simulink model "DualBuckPPS22016"  (R2024b)
settings: Solver=ode45  StartTime=0.0  StopTime=0.5  RelTol=1e-3
model workspace (MAT data in the model file):
  D = 50
  T = 0.0333333333333
undefined symbols (not defined in the file): D_T_DOWN_Given, D_T_UP_Given, DiscIntNeverNeededParam, P, T_pulse, TP
libraries: spsOnDelayLib x30, dspsnks4 x12, dspfdesign x11, spsCurrentMeasurementLib x11, spsSeriesRLCBranchLib x6, spsMosfetLib x4, slpidlib x4, spsVoltageMeasurementLib x4, simulink x3, spsControlledCurrentSourceLib x1, spsDCVoltageSourceLib x1, spspowerguiLib x1
(part 1 of 2)
settings Model: SimulationMode=accelerator  Creator=10474  LastModifiedBy=admin
settings SolverCC: AlgebraicLoopSolver=TrustRegion
settings OptimizationCC: ReuseModelBlockBuffer=off
settings DebuggingCC: UnconnectedInputMsg=warning  UnconnectedOutputMsg=warning  UnconnectedLineMsg=warning  ArithmeticOperatorsInVariantConditions=warning
settings ModelReferenceCC: EnableRefExpFcnMdlSchedulingChecks=on
settings SFSimCC: CustomCodeUndefinedFunction=UseInterfaceOnly
settings RTWCC: GPUComputeCapability=3.5
settings CodeAppCC: StateflowObjectComments=on

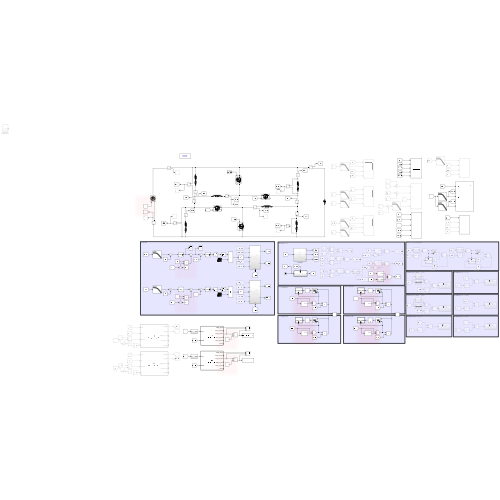
[thumbnail: Simulink's stored preview of the top-level diagram]
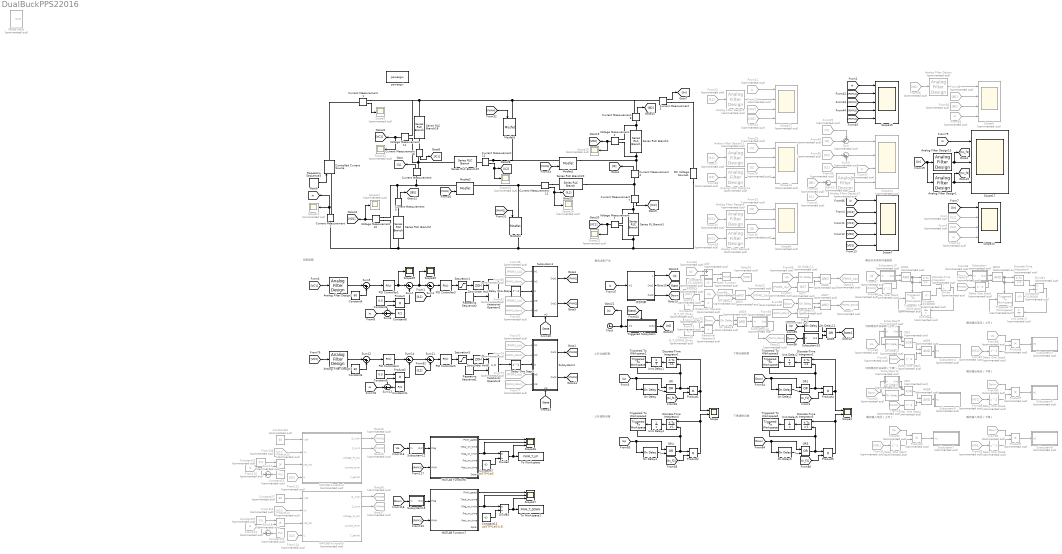
== system DualBuckPPS22016 ==
  note: 控制回路
  note: 上升尖峰获取
  note: 上升滤除尖峰
  note: 下降尖峰获取
  note: 下降滤除尖峰
  note: 瞬态输出电压（上升）
  note: 切回稳态开关采样（上升）
  note: 瞬态输入电压（上升）
  note: 瞬态输入电压（下降）
  note: 瞬态开关序列均值获取
  note: 瞬态输出电压（下降）
  note: 切回稳态开关采样（下降）
  note: 瞬态波形产生
  AND{1..8} (8 alike) : Logic  Commented=on  IconShape=distinctive  AllPortsSameDT=off  OutDataTypeStr=boolean
  AND9 : Logic  Operator=OR  IconShape=distinctive  AllPortsSameDT=off  OutDataTypeStr=boolean
  Add : Sum  Commented=on  Inputs=+-
  Analog Filter Design{,5..6,9..12} (7 alike) : dspfdesign/Analog Filter Design  Commented=on  method=Butterworth  filttype=Lowpass  N=8  Wlo=2*pi*5000  Whi=80  Rp=2  Rs=40
  Analog Filter Design1 : dspfdesign/Analog Filter Design  method=Butterworth  filttype=Lowpass  N=2  Wlo=2*pi*2500  Whi=80  Rp=2  Rs=40
  Analog Filter Design13 : dspfdesign/Analog Filter Design  method=Butterworth  filttype=Lowpass  N=2  Wlo=2*pi*10000  Whi=80  Rp=2  Rs=40
  Analog Filter Design2 : dspfdesign/Analog Filter Design  method=Butterworth  filttype=Lowpass  N=1  Wlo=10  Whi=80  Rp=2  Rs=40
  Analog Filter Design3 : dspfdesign/Analog Filter Design  method=Butterworth  filttype=Lowpass  N=1  Wlo=10  Whi=80  Rp=2  Rs=40
  Clock : Clock
  Constant : Constant  Commented=on  Value=1/100000
  Constant1 : Constant  Commented=on  Value=1/100000
  Constant10 : Constant  Commented=on  Value=D_T_DOWN_Given
  Constant11 : Constant  Value=P/2
  Constant12 : Constant  Value=ceil(TP*1e5-0.5)
  Constant2 : Constant  Commented=on  Value=D_T_UP_Given
  Constant22 : Constant  Commented=on  Value=0.5
  Constant23 : Constant  Commented=on  Value=P/2
  Constant24 : Constant  Commented=on  Value=60
  Constant25 : Constant  Commented=on  Value=0.5
  Constant26 : Constant  Commented=on  Value=P/2
  Constant27 : Constant  Commented=on  Value=60
  Constant3 : Constant  Value=60
  Constant4 : Constant  Value=60
  Constant5 : Constant  Commented=on  Value=1/100000
  Constant6 : Constant  Value=0.5
  Constant7 : Constant  Value=ceil(TP*1e5)
  Constant8 : Constant  Value=P/2
  Constant9 : Constant  Value=0.5
  Controlled Current Source : spsControlledCurrentSourceLib/Controlled Current Source  Initialize=on  Source_Type=DC  Amplitude=0  Phase=0  Frequency=0  Measurements=None
  Current Measurement{,1..8,11..12} (11 alike) : spsCurrentMeasurementLib/Current Measurement  PhasorSimulation=off  OutputType=Complex  PSBequivalent=0
  DC Voltage Source1 : spsDCVoltageSourceLib/DC Voltage Source  Amplitude=270  Measurements=None
  Delay One Step : Delay  DelayLength=1
  Delay One Step1 : Delay  Commented=on
  Delay One Step{2..3,5..8} (6 alike) : Delay  Commented=on  DelayLength=1
  Delay One Step4 : Delay  Commented=on
  Delay One Step9 : Delay  DelayLength=1
  Discrete-Time Integrator : DiscreteIntegrator  Commented=on  ExternalReset=falling  SampleTime=-1  ICPrevOutput=DiscIntNeverNeededParam  ICPrevScaledInput=DiscIntNeverNeededParam
  Discrete-Time Integrator{1..2,4..5} (4 alike) : DiscreteIntegrator  ExternalReset=falling  SampleTime=-1  ICPrevOutput=DiscIntNeverNeededParam  ICPrevScaledInput=DiscIntNeverNeededParam
  Discrete-Time Integrator3 : DiscreteIntegrator  Commented=on  ExternalReset=falling  SampleTime=-1  ICPrevOutput=DiscIntNeverNeededParam  ICPrevScaledInput=DiscIntNeverNeededParam
  Divide : Product  Commented=on  Inputs=*/
  Divide1 : Product  Commented=on  Inputs=*/
  Divide2 : Product  Inputs=*/
  Divide3 : Product  Inputs=*/
  From{,22,27,36,111} (5 alike) : From  Commented=on  GotoTag=IL1
  From{10,55,61,66} (4 alike) : From  Commented=on  GotoTag=PWM1
  From109 : From  Commented=on  GotoTag=VC1
  From{14,21,37,39,110,113} (6 alike) : From  Commented=on  GotoTag=io  TagVisibility=global
  From112 : From  Commented=on  GotoTag=VC2
  From{9,28,35,114} (4 alike) : From  Commented=on  GotoTag=IL2
  From{15,25,29,41} (4 alike) : From  Commented=on  GotoTag=I1
  From16 : From  Commented=on  GotoTag=I2
  From17 : From  Commented=on  GotoTag=IC1
  From18 : From  Commented=on  GotoTag=IC2
  From23 : From  Commented=on  GotoTag=VC2
  From24 : From  Commented=on  GotoTag=VG2
  From26 : From  Commented=on  GotoTag=I2
  From34 : From  Commented=on  GotoTag=I2
  From38 : From  Commented=on  GotoTag=IB2
  From40 : From  Commented=on  GotoTag=IB1
  From46 : From  Commented=on  GotoTag=IB1
  From48 : From  Commented=on  GotoTag=IB1
  From49 : From  Commented=on  GotoTag=PWM1_Up
  From50 : From  Commented=on  GotoTag=PWM1_Down
  From51 : From  Commented=on  GotoTag=PWM2_Up
  From{56,67..69,89,92} (6 alike) : From  Commented=on  GotoTag=Up  TagVisibility=global
  From57 : From  Commented=on  GotoTag=PWM1_Up
  From{58,60,72,82,90,94} (6 alike) : From  Commented=on  GotoTag=Down  TagVisibility=global
  From59 : From  Commented=on  GotoTag=PWM1_Down
  From62 : From  Commented=on  GotoTag=PWM2_Down
  From63 : From  Commented=on  GotoTag=t0
  From65 : From  Commented=on  GotoTag=t
  From70 : From  Commented=on  GotoTag=PWM1_Up
  From71 : From  Commented=on  GotoTag=MW
  From73 : From  Commented=on  GotoTag=MW
  From74 : From  Commented=on  GotoTag=PWM1_Down
  From75 : From  Commented=on  GotoTag=PWM2_Up
  From77 : From  Commented=on  GotoTag=PWM2_Down
  From87 : From  Commented=on  GotoTag=VC1
  From88 : From  Commented=on  GotoTag=VC1
  From91 : From  Commented=on  GotoTag=VG1
  From93 : From  Commented=on  GotoTag=VG1
  Goto16 : Goto  Commented=on  GotoTag=PWM2_Up
  Goto17 : Goto  Commented=on  GotoTag=PWM2_Down
  Goto22 : Goto  Commented=on  GotoTag=PWM1_Down
  Goto23 : Goto  Commented=on  GotoTag=PWM1_Up
  Goto24 : Goto  Commented=on  GotoTag=MW
  Goto25 : Goto  Commented=on  GotoTag=PWM1
  Goto26 : Goto  Commented=on  GotoTag=PWM2
  Goto36 : Goto  Commented=on  GotoTag=PWM3
  Goto37 : Goto  Commented=on  GotoTag=PWM4
  MATLAB Function4 : MATLAB Function  Commented=on  TreatAsAtomicUnit=on
  MATLAB Function5 : MATLAB Function  Commented=on  TreatAsAtomicUnit=on
  MATLAB Function6 : MATLAB Function  TreatAsAtomicUnit=on
  MATLAB Function7 : MATLAB Function  TreatAsAtomicUnit=on
  Math Function : Math  Commented=on  Operator=mod
  Mosfet{1..4} (4 alike) : spsMosfetLib/Mosfet  Ron=53e-3  Lon=0  Rd=0.001  Vfd=2  IC=0  Rs=1e5  Cs=inf  Measurements=on
  NOT7 : Logic  Commented=on  Operator=NOT  IconShape=distinctive  AllPortsSameDT=off  OutDataTypeStr=boolean
  NOT8 : Logic  Commented=on  Operator=NOT  IconShape=distinctive  AllPortsSameDT=off  OutDataTypeStr=boolean
  OR{,1,4..5} (4 alike) : Logic  Operator=OR  IconShape=distinctive  AllPortsSameDT=off  OutDataTypeStr=boolean
  OR2 : Logic  Commented=on  Operator=XOR  IconShape=distinctive  AllPortsSameDT=off  OutDataTypeStr=boolean
  OR3 : Logic  Commented=on  Operator=XOR  IconShape=distinctive  AllPortsSameDT=off  OutDataTypeStr=boolean
  On Delay{,1,4..5} (4 alike) : spsOnDelayLib/On Delay  DelayType=Off delay  delay=TP  ic=0  Ts=0
  On Delay10 : spsOnDelayLib/On Delay  Commented=on  DelayType=Off delay  delay=ceil((TP-(ceil(TP*1e5)*1e-5-TP))*1e5)*1e-5-(TP-(ceil(TP*1e5)*1e-5-TP))  ic=0  Ts=0
  On Delay11 : spsOnDelayLib/On Delay  DelayType=Off delay  delay=ceil(TP*1e5)*1e-5-TP  ic=0  Ts=0
  On Delay12 : spsOnDelayLib/On Delay  Commented=on  DelayType=Off delay  delay=ceil(TP*1e5)*1e-5-TP  ic=0  Ts=0
  On Delay2 : spsOnDelayLib/On Delay  Commented=on  DelayType=Off delay  delay=ceil(TP*1e5)*1e-5-TP  ic=0  Ts=0
  On Delay3 : spsOnDelayLib/On Delay  Commented=on  DelayType=Off delay  delay=30e-6  ic=0  Ts=0
  On Delay8 : spsOnDelayLib/On Delay  Commented=on  DelayType=Off delay  delay=ceil((TP-(ceil(TP*1e5)*1e-5-TP))*1e5)*1e-5-(TP-(ceil(TP*1e5)*1e-5-TP))  ic=0  Ts=0
  On Delay9 : spsOnDelayLib/On Delay  Commented=on  DelayType=Off delay  delay=30e-6  ic=0  Ts=0
  PID Controller1 : slpidlib/PID Controller  Controller=PI  Form=Parallel  TimeDomain=Discrete-time  UseExternalTs=off  SampleTime=-1  IntegratorMethod=Forward Euler  FilterMethod=Forward Euler  ControllerParametersSource=internal  P=0.15  I=0.5  UseKiTs=off  D=0  UseExternalDerivativeSource=off  N=100  UseFilter=on  TunerSelectOption=Transfer Function Based (PID Tuner App)  InitialConditionSource=internal  InitialConditionForIntegrator=0  InitialConditionForFilter=0  DifferentiatorICPrevScaledInput=0  ExternalReset=none  TrackingMode=off  Kt=1  LimitOutput=on  SatLimitsSource=internal  UpperSaturationLimit=10  LowerSaturationLimit=-10  LinearizeAsGain=on  AntiWindupMode=none  Kb=1  LimitIntegrator=off  UpperIntegratorSaturationLimit=inf  LowerIntegratorSaturationLimit=-inf  POutMin=[]  POutMax=[]  IOutMin=[]  IOutMax=[]  DOutMin=[]  DOutMax=[]  NOutMin=[]  NOutMax=[]  SumOutMin=[]  SumOutMax=[]  SaturationOutMin=[]  SaturationOutMax=[]  PParamMin=[]  PParamMax=[]  IParamMin=[]  IParamMax=[]  DParamMin=[]  DParamMax=[]  NParamMin=[]  NParamMax=[]  KbParamMin=[]  KbParamMax=[]  KtParamMin=[]  KtParamMax=[]  KbOutMin=[]  KbOutMax=[]  KtOutMin=[]  KtOutMax=[]  IntegratorOutMin=[]  IntegratorOutMax=[]  FilterOutMin=[]  FilterOutMax=[]  SumI1OutMin=[]  SumI1OutMax=[]  SumI2OutMin=[]  SumI2OutMax=[]  SumI3OutMin=[]  SumI3OutMax=[]  SumI4OutMin=[]  SumI4OutMax=[]  SumDOutMin=[]  SumDOutMax=[]  DifferentiatorOutMin=[]  DifferentiatorOutMax=[]  FilterDiffOutCoefMin=[]  FilterDiffOutCoefMax=[]  ReciprocalOutMin=[]  ReciprocalOutMax=[]  SumDenOutMin=[]  SumDenOutMax=[]  SumNumOutMin=[]  SumNumOutMax=[]  DivideOutMin=[]  DivideOutMax=[]  UdiffTsProdOutMin=[]  UdiffTsProdOutMax=[]  NTsProdOutMin=[]  NTsProdOutMax=[]  UintegralTsProdOutMin=[]  UintegralTsProdOutMax=[]  UngainTsProdOutMin=[]  UngainTsProdOutMax=[]  ClampingZeroOutDataTypeStr=Inherit: Inherit via back propagation  ClampingZeroOutMin=[]  ClampingZeroOutMax=[]  FilterDenConstantOutDataTypeStr=Inherit: Inherit via back propagation  FilterDenConstantOutMin=[]  FilterDenConstantOutMax=[]  PCopyOutDataTypeStr=Inherit: Inherit via back propagation  PCopyOutMin=[]  PCopyOutMax=[]  NCopyOutDataTypeStr=Inherit: Inherit via back propagation  NCopyOutMin=[]  NCopyOutMax=[]  IntegratorContinuousStateAttributes=''  IntegratorStateMustResolveToSignalObject=off  IntegratorRTWStateStorageClass=Auto  FilterContinuousStateAttributes=''  FilterStateMustResolveToSignalObject=off  FilterRTWStateStorageClass=Auto  ParallelPVariant=InternalParameters  IdealPVariant=Disabled  IVariant=InternalParameters  DVariant=Disabled  IntegratorVariant=Discrete  SatVariant=Enabled  AWVariant=Passthrough  PCopyVariant=Disabled  TRVariant=Disabled  FdbkBlocksVariant=Forward  IdealPFdbkVariant=Disabled  SatFdbkVariant=Disabled  DerivativeFilterVariant=Disabled  NVariant=Disabled  NCopyVariant=Disabled_SignalSpec  FilterICVariant=Disabled  IntegratorICVariant=InternalICs  ExternalResetVariant=Disabled  TRSumVariant=Passthrough  SumFdbkVariant=Disabled  SumVariant=Sum_PI  TsampFilterVariant=InternalTs  TsampNgainVariant=Passthrough  TsampIntegralVariant=Disabled_SignalSpec  ExternalSaturationOutDataTypeStr=Inherit: Same as second input  DerivativeSourceVariant=Disabled  PreIntVariant=InternalPreInt
  PID Controller3 : slpidlib/PID Controller  Controller=PI  Form=Parallel  TimeDomain=Discrete-time  UseExternalTs=off  SampleTime=-1  IntegratorMethod=Forward Euler  FilterMethod=Forward Euler  ControllerParametersSource=internal  P=0.2  I=2  UseKiTs=off  D=0  UseExternalDerivativeSource=off  N=100  UseFilter=on  TunerSelectOption=Transfer Function Based (PID Tuner App)  InitialConditionSource=internal  InitialConditionForIntegrator=0  InitialConditionForFilter=0  DifferentiatorICPrevScaledInput=0  ExternalReset=none  TrackingMode=off  Kt=1  LimitOutput=on  SatLimitsSource=internal  UpperSaturationLimit=0.98  LowerSaturationLimit=0  LinearizeAsGain=on  AntiWindupMode=none  Kb=1  LimitIntegrator=off  UpperIntegratorSaturationLimit=inf  LowerIntegratorSaturationLimit=-inf  POutMin=[]  POutMax=[]  IOutMin=[]  IOutMax=[]  DOutMin=[]  DOutMax=[]  NOutMin=[]  NOutMax=[]  SumOutMin=[]  SumOutMax=[]  SaturationOutMin=[]  SaturationOutMax=[]  PParamMin=[]  PParamMax=[]  IParamMin=[]  IParamMax=[]  DParamMin=[]  DParamMax=[]  NParamMin=[]  NParamMax=[]  KbParamMin=[]  KbParamMax=[]  KtParamMin=[]  KtParamMax=[]  KbOutMin=[]  KbOutMax=[]  KtOutMin=[]  KtOutMax=[]  IntegratorOutMin=[]  IntegratorOutMax=[]  FilterOutMin=[]  FilterOutMax=[]  SumI1OutMin=[]  SumI1OutMax=[]  SumI2OutMin=[]  SumI2OutMax=[]  SumI3OutMin=[]  SumI3OutMax=[]  SumI4OutMin=[]  SumI4OutMax=[]  SumDOutMin=[]  SumDOutMax=[]  DifferentiatorOutMin=[]  DifferentiatorOutMax=[]  FilterDiffOutCoefMin=[]  FilterDiffOutCoefMax=[]  ReciprocalOutMin=[]  ReciprocalOutMax=[]  SumDenOutMin=[]  SumDenOutMax=[]  SumNumOutMin=[]  SumNumOutMax=[]  DivideOutMin=[]  DivideOutMax=[]  UdiffTsProdOutMin=[]  UdiffTsProdOutMax=[]  NTsProdOutMin=[]  NTsProdOutMax=[]  UintegralTsProdOutMin=[]  UintegralTsProdOutMax=[]  UngainTsProdOutMin=[]  UngainTsProdOutMax=[]  ClampingZeroOutDataTypeStr=Inherit: Inherit via back propagation  ClampingZeroOutMin=[]  ClampingZeroOutMax=[]  FilterDenConstantOutDataTypeStr=Inherit: Inherit via back propagation  FilterDenConstantOutMin=[]  FilterDenConstantOutMax=[]  PCopyOutDataTypeStr=Inherit: Inherit via back propagation  PCopyOutMin=[]  PCopyOutMax=[]  NCopyOutDataTypeStr=Inherit: Inherit via back propagation  NCopyOutMin=[]  NCopyOutMax=[]  IntegratorContinuousStateAttributes=''  IntegratorStateMustResolveToSignalObject=off  IntegratorRTWStateStorageClass=Auto  FilterContinuousStateAttributes=''  FilterStateMustResolveToSignalObject=off  FilterRTWStateStorageClass=Auto  ParallelPVariant=InternalParameters  IdealPVariant=Disabled  IVariant=InternalParameters  DVariant=Disabled  IntegratorVariant=Discrete  SatVariant=Enabled  AWVariant=Passthrough  PCopyVariant=Disabled  TRVariant=Disabled  FdbkBlocksVariant=Forward  IdealPFdbkVariant=Disabled  SatFdbkVariant=Disabled  DerivativeFilterVariant=Disabled  NVariant=Disabled  NCopyVariant=Disabled_SignalSpec  FilterICVariant=Disabled  IntegratorICVariant=InternalICs  ExternalResetVariant=Disabled  TRSumVariant=Passthrough  SumFdbkVariant=Disabled  SumVariant=Sum_PI  TsampFilterVariant=InternalTs  TsampNgainVariant=Passthrough  TsampIntegralVariant=Disabled_SignalSpec  ExternalSaturationOutDataTypeStr=Inherit: Same as second input  DerivativeSourceVariant=Disabled  PreIntVariant=InternalPreInt
  PID Controller4 : slpidlib/PID Controller  Controller=PI  Form=Parallel  TimeDomain=Discrete-time  UseExternalTs=off  SampleTime=-1  IntegratorMethod=Forward Euler  FilterMethod=Forward Euler  ControllerParametersSource=internal  P=0.15  I=0.5  UseKiTs=off  D=0  UseExternalDerivativeSource=off  N=100  UseFilter=on  TunerSelectOption=Transfer Function Based (PID Tuner App)  InitialConditionSource=internal  InitialConditionForIntegrator=0  InitialConditionForFilter=0  DifferentiatorICPrevScaledInput=0  ExternalReset=none  TrackingMode=off  Kt=1  LimitOutput=off  SatLimitsSource=internal  UpperSaturationLimit=1  LowerSaturationLimit=-1  LinearizeAsGain=on  AntiWindupMode=none  Kb=1  LimitIntegrator=off  UpperIntegratorSaturationLimit=inf  LowerIntegratorSaturationLimit=-inf  POutMin=[]  POutMax=[]  IOutMin=[]  IOutMax=[]  DOutMin=[]  DOutMax=[]  NOutMin=[]  NOutMax=[]  SumOutMin=[]  SumOutMax=[]  SaturationOutMin=[]  SaturationOutMax=[]  PParamMin=[]  PParamMax=[]  IParamMin=[]  IParamMax=[]  DParamMin=[]  DParamMax=[]  NParamMin=[]  NParamMax=[]  KbParamMin=[]  KbParamMax=[]  KtParamMin=[]  KtParamMax=[]  KbOutMin=[]  KbOutMax=[]  KtOutMin=[]  KtOutMax=[]  IntegratorOutMin=[]  IntegratorOutMax=[]  FilterOutMin=[]  FilterOutMax=[]  SumI1OutMin=[]  SumI1OutMax=[]  SumI2OutMin=[]  SumI2OutMax=[]  SumI3OutMin=[]  SumI3OutMax=[]  SumI4OutMin=[]  SumI4OutMax=[]  SumDOutMin=[]  SumDOutMax=[]  DifferentiatorOutMin=[]  DifferentiatorOutMax=[]  FilterDiffOutCoefMin=[]  FilterDiffOutCoefMax=[]  ReciprocalOutMin=[]  ReciprocalOutMax=[]  SumDenOutMin=[]  SumDenOutMax=[]  SumNumOutMin=[]  SumNumOutMax=[]  DivideOutMin=[]  DivideOutMax=[]  UdiffTsProdOutMin=[]  UdiffTsProdOutMax=[]  NTsProdOutMin=[]  NTsProdOutMax=[]  UintegralTsProdOutMin=[]  UintegralTsProdOutMax=[]  UngainTsProdOutMin=[]  UngainTsProdOutMax=[]  ClampingZeroOutDataTypeStr=Inherit: Inherit via back propagation  ClampingZeroOutMin=[]  ClampingZeroOutMax=[]  FilterDenConstantOutDataTypeStr=Inherit: Inherit via back propagation  FilterDenConstantOutMin=[]  FilterDenConstantOutMax=[]  PCopyOutDataTypeStr=Inherit: Inherit via back propagation  PCopyOutMin=[]  PCopyOutMax=[]  NCopyOutDataTypeStr=Inherit: Inherit via back propagation  NCopyOutMin=[]  NCopyOutMax=[]  IntegratorContinuousStateAttributes=''  IntegratorStateMustResolveToSignalObject=off  IntegratorRTWStateStorageClass=Auto  FilterContinuousStateAttributes=''  FilterStateMustResolveToSignalObject=off  FilterRTWStateStorageClass=Auto  ParallelPVariant=InternalParameters  IdealPVariant=Disabled  IVariant=InternalParameters  DVariant=Disabled  IntegratorVariant=Discrete  SatVariant=Disabled  AWVariant=Passthrough  PCopyVariant=Disabled  TRVariant=Disabled  FdbkBlocksVariant=Forward  IdealPFdbkVariant=Disabled  SatFdbkVariant=Disabled  DerivativeFilterVariant=Disabled  NVariant=Disabled  NCopyVariant=Disabled_SignalSpec  FilterICVariant=Disabled  IntegratorICVariant=InternalICs  ExternalResetVariant=Disabled  TRSumVariant=Passthrough  SumFdbkVariant=Disabled  SumVariant=Sum_PI  TsampFilterVariant=InternalTs  TsampNgainVariant=Passthrough  TsampIntegralVariant=Disabled_SignalSpec  ExternalSaturationOutDataTypeStr=Inherit: Same as second input  DerivativeSourceVariant=Disabled  PreIntVariant=InternalPreInt
  PID Controller5 : slpidlib/PID Controller  Controller=PI  Form=Parallel  TimeDomain=Discrete-time  UseExternalTs=off  SampleTime=-1  IntegratorMethod=Forward Euler  FilterMethod=Forward Euler  ControllerParametersSource=internal  P=0.2  I=2  UseKiTs=off  D=0  UseExternalDerivativeSource=off  N=100  UseFilter=on  TunerSelectOption=Transfer Function Based (PID Tuner App)  InitialConditionSource=internal  InitialConditionForIntegrator=0  InitialConditionForFilter=0  DifferentiatorICPrevScaledInput=0  ExternalReset=none  TrackingMode=off  Kt=1  LimitOutput=on  SatLimitsSource=internal  UpperSaturationLimit=0.98  LowerSaturationLimit=0  LinearizeAsGain=on  AntiWindupMode=none  Kb=1  LimitIntegrator=off  UpperIntegratorSaturationLimit=inf  LowerIntegratorSaturationLimit=-inf  POutMin=[]  POutMax=[]  IOutMin=[]  IOutMax=[]  DOutMin=[]  DOutMax=[]  NOutMin=[]  NOutMax=[]  SumOutMin=[]  SumOutMax=[]  SaturationOutMin=[]  SaturationOutMax=[]  PParamMin=[]  PParamMax=[]  IParamMin=[]  IParamMax=[]  DParamMin=[]  DParamMax=[]  NParamMin=[]  NParamMax=[]  KbParamMin=[]  KbParamMax=[]  KtParamMin=[]  KtParamMax=[]  KbOutMin=[]  KbOutMax=[]  KtOutMin=[]  KtOutMax=[]  IntegratorOutMin=[]  IntegratorOutMax=[]  FilterOutMin=[]  FilterOutMax=[]  SumI1OutMin=[]  SumI1OutMax=[]  SumI2OutMin=[]  SumI2OutMax=[]  SumI3OutMin=[]  SumI3OutMax=[]  SumI4OutMin=[]  SumI4OutMax=[]  SumDOutMin=[]  SumDOutMax=[]  DifferentiatorOutMin=[]  DifferentiatorOutMax=[]  FilterDiffOutCoefMin=[]  FilterDiffOutCoefMax=[]  ReciprocalOutMin=[]  ReciprocalOutMax=[]  SumDenOutMin=[]  SumDenOutMax=[]  SumNumOutMin=[]  SumNumOutMax=[]  DivideOutMin=[]  DivideOutMax=[]  UdiffTsProdOutMin=[]  UdiffTsProdOutMax=[]  NTsProdOutMin=[]  NTsProdOutMax=[]  UintegralTsProdOutMin=[]  UintegralTsProdOutMax=[]  UngainTsProdOutMin=[]  UngainTsProdOutMax=[]  ClampingZeroOutDataTypeStr=Inherit: Inherit via back propagation  ClampingZeroOutMin=[]  ClampingZeroOutMax=[]  FilterDenConstantOutDataTypeStr=Inherit: Inherit via back propagation  FilterDenConstantOutMin=[]  FilterDenConstantOutMax=[]  PCopyOutDataTypeStr=Inherit: Inherit via back propagation  PCopyOutMin=[]  PCopyOutMax=[]  NCopyOutDataTypeStr=Inherit: Inherit via back propagation  NCopyOutMin=[]  NCopyOutMax=[]  IntegratorContinuousStateAttributes=''  IntegratorStateMustResolveToSignalObject=off  IntegratorRTWStateStorageClass=Auto  FilterContinuousStateAttributes=''  FilterStateMustResolveToSignalObject=off  FilterRTWStateStorageClass=Auto  ParallelPVariant=InternalParameters  IdealPVariant=Disabled  IVariant=InternalParameters  DVariant=Disabled  IntegratorVariant=Discrete  SatVariant=Enabled  AWVariant=Passthrough  PCopyVariant=Disabled  TRVariant=Disabled  FdbkBlocksVariant=Forward  IdealPFdbkVariant=Disabled  SatFdbkVariant=Disabled  DerivativeFilterVariant=Disabled  NVariant=Disabled  NCopyVariant=Disabled_SignalSpec  FilterICVariant=Disabled  IntegratorICVariant=InternalICs  ExternalResetVariant=Disabled  TRSumVariant=Passthrough  SumFdbkVariant=Disabled  SumVariant=Sum_PI  TsampFilterVariant=InternalTs  TsampNgainVariant=Passthrough  TsampIntegralVariant=Disabled_SignalSpec  ExternalSaturationOutDataTypeStr=Inherit: Same as second input  DerivativeSourceVariant=Disabled  PreIntVariant=InternalPreInt
  Product{,1..5} (6 alike) : Product
  Product{6..9,13..14} (6 alike) : Product  Commented=on
  Relational Operator : RelationalOperator  Commented=on  Operator=<  OutDataTypeStr=boolean  RndMeth=Simplest  InputSameDT=off
  Relational Operator2 : RelationalOperator  OutDataTypeStr=boolean  RndMeth=Simplest  InputSameDT=off
  Relational Operator3 : RelationalOperator  OutDataTypeStr=boolean  RndMeth=Simplest  InputSameDT=off
  Relational Operator5 : RelationalOperator  Commented=on  Operator=<  OutDataTypeStr=boolean  RndMeth=Simplest  InputSameDT=off
  Repeating Sequence1 : simulink/Sources/Repeating Sequence  rep_seq_t=[0 1/100000]  rep_seq_y=[0 1]
  Repeating Sequence2 : simulink/Sources/Repeating Sequence  rep_seq_t=[0 1/100000]  rep_seq_y=[0 1]
  Repeating Sequence3 : simulink/Sources/Repeating Sequence  rep_seq_t=[0 TP T_pulse/2+TP T_pulse/2+2*TP T_pulse]  rep_seq_y=[0 P P 0 0]
  Saturation1 : Saturate  UpperLimit=0.98  LowerLimit=0
  Saturation3 : Saturate  UpperLimit=0.98  LowerLimit=0
  Scope : Scope  NumInputPorts=2
  Scope1 : Scope  NumInputPorts=2
  Scope10 : Scope  NumInputPorts=4
  Scope{9,11,16,18..19,21..23} (8 alike) : Scope  Commented=on
  Scope{6,8,12..14} (5 alike) : Scope  Commented=on  NumInputPorts=4
  Scope15 : Scope  NumInputPorts=5
  Scope17 : Scope  NumInputPorts=3
  Scope26 : Scope  NumInputPorts=3
  Scope27 : Scope  NumInputPorts=3
  Scope29 : Scope
  Scope30 : Scope
  Scope7 : Scope  NumInputPorts=5
  Series RL Branch1 : spsSeriesRLCBranchLib/Series RLC Branch  LConnTagsString=__new0  RConnTagsString=__new0  BranchType=RC  Resistance=0.001  Inductance=1e-3  SetiL0=off  InitialCurrent=0  Capacitance=1e-6  Setx0=on  InitialVoltage=12  Measurements=None
  Series RLC Branch1 : spsSeriesRLCBranchLib/Series RLC Branch  LConnTagsString=__new0  RConnTagsString=__new0  BranchType=RC  Resistance=0.001  Inductance=1e-3  SetiL0=off  InitialCurrent=0  Capacitance=2.48e-3  Setx0=on  InitialVoltage=12  Measurements=None
  Series RLC Branch18 : spsSeriesRLCBranchLib/Series RLC Branch  LConnTagsString=__new0  RConnTagsString=__new0  BranchType=RC  Resistance=0.001  Inductance=1e-3  SetiL0=off  InitialCurrent=0  Capacitance=1e-6  Setx0=on  InitialVoltage=12  Measurements=None
  Series RLC Branch19 : spsSeriesRLCBranchLib/Series RLC Branch  LConnTagsString=__new0  RConnTagsString=__new0  BranchType=L  Resistance=0.01  Inductance=260e-6  SetiL0=off  InitialCurrent=15  Capacitance=1e-3  Setx0=off  InitialVoltage=0  Measurements=None
  Series RLC Branch2 : spsSeriesRLCBranchLib/Series RLC Branch  LConnTagsString=__new0  RConnTagsString=__new0  BranchType=RC  Resistance=0.2  Inductance=1e-3  SetiL0=off  InitialCurrent=0  Capacitance=2.48e-3  Setx0=on  InitialVoltage=12  Measurements=None
  Series RLC Branch20 : spsSeriesRLCBranchLib/Series RLC Branch  LConnTagsString=__new0  RConnTagsString=__new0  BranchType=L  Resistance=0.01  Inductance=260e-6  SetiL0=off  InitialCurrent=5  Capacitance=1e-3  Setx0=off  InitialVoltage=0  Measurements=None
  Subsystem : Subsystem  Commented=on
  Subsystem1 : Subsystem
      settings: PortSchema="{\"entries\":[{\"content\":{\"sides\":[{\"content\":{\"connectorIds\":[\"In1\",\"In2\",\"In3\",\"In4\",\"In5\"]},\"type\":\"ConnectorPlacement.EquallySpacedRectSide\",\"uuid\":\"12f56cea-dd87-479d-8ac5-f677a0a856ab\"},{\"content\":{\"connectorIds\":[\"Out1\",\"Out2\"],\"side\":\"RIGHT\"},\"type\":\"ConnectorPlacement.EquallySpacedRectSide\",\"uuid\":\"93daadb0-c8ef-4d9e-87ae-a550f970c223\"},{\"content\":{\"side\":\"TOP\"},\"type\":\"ConnectorPlacement.EquallySpacedRectSide\",\"uuid\":\"18f26d28-3d48-45f0-84e1-51e7663a8b99\"},{\"content\":{\"connectorIds\":[\"In6\"],\"side\":\"BOTTOM\"},\"type\":\"ConnectorPlacement.EquallySpacedRectSide\",\"uuid\":\"53ae5f66-9a34-49e2-9ad8-502cdcf805c1\"}]},\"type\":\"ConnectorPlacement.EquallySpacedConnector\",\"uuid\":\"751889f7-46a5-4d64-ba57-d2d7ffe777e8\"}],\"packageUris\":[\"http://schema.mathworks.com/mf0/Connector/R2020b\"],\"version\":\"1.0\"}"
  Subsystem10 : Subsystem  Commented=on
  Subsystem11 : Subsystem  Commented=on
  Subsystem12 : Subsystem
  Subsystem13 : Subsystem
  Subsystem14 : Subsystem  Commented=on
  Subsystem15 : Subsystem
  Subsystem2 : Subsystem
      settings: PortSchema="{\"entries\":[{\"content\":{\"sides\":[{\"content\":{\"connectorIds\":[\"In1\",\"In2\",\"In3\",\"In4\",\"In5\"]},\"type\":\"ConnectorPlacement.EquallySpacedRectSide\",\"uuid\":\"12f56cea-dd87-479d-8ac5-f677a0a856ab\"},{\"content\":{\"connectorIds\":[\"Out1\",\"Out2\"],\"side\":\"RIGHT\"},\"type\":\"ConnectorPlacement.EquallySpacedRectSide\",\"uuid\":\"93daadb0-c8ef-4d9e-87ae-a550f970c223\"},{\"content\":{\"side\":\"TOP\"},\"type\":\"ConnectorPlacement.EquallySpacedRectSide\",\"uuid\":\"18f26d28-3d48-45f0-84e1-51e7663a8b99\"},{\"content\":{\"connectorIds\":[\"In6\"],\"side\":\"BOTTOM\"},\"type\":\"ConnectorPlacement.EquallySpacedRectSide\",\"uuid\":\"53ae5f66-9a34-49e2-9ad8-502cdcf805c1\"}]},\"type\":\"ConnectorPlacement.EquallySpacedConnector\",\"uuid\":\"751889f7-46a5-4d64-ba57-d2d7ffe777e8\"}],\"packageUris\":[\"http://schema.mathworks.com/mf0/Connector/R2020b\"],\"version\":\"1.0\"}"
  Subsystem3 : Subsystem  Commented=on
  Subsystem4 : Subsystem  Commented=on
  Subsystem5 : Subsystem  Commented=on
  Subsystem6 : Subsystem  Commented=on
  Subsystem7 : Subsystem  Commented=on
  Subsystem8 : Subsystem  Commented=on
  Subsystem9 : Subsystem  Commented=on
  Sum : Sum  Commented=on  Inputs=++|
  Sum{1,7,11,14} (4 alike) : Sum  Inputs=|+-
  Sum10 : Sum  Commented=on  Inputs=|+-
  Sum12 : Sum  Inputs=|-+
  Sum13 : Sum  Inputs=+-
  Sum17 : Sum  Commented=on  Inputs=+-
  Sum18 : Sum  Commented=on  Inputs=+-
  Sum5 : Sum  Inputs=|-+
  Sum6 : Sum  Inputs=+-
  Sum9 : Sum  Commented=on  Inputs=|++
  To Workspace : ToWorkspace  VariableName=PWM_T_UP  SampleTime=1e-4
      settings: Save2DSignal=2-D array (concatenate along first dimension)
  To Workspace1 : ToWorkspace  VariableName=PWM_T_DOWN  SampleTime=1e-4
      settings: Save2DSignal=2-D array (concatenate along first dimension)
  Triggered Subsystem : Subsystem  TreatAsAtomicUnit=on
  Triggered To Workspace : dspsnks4/Triggered To Workspace  Commented=on  TriggerType=Falling edge  VariableName=PWM_T_UP  Buffer=1000  Save2DMode=2-D array (concatenate along first dimension)
      settings: FixptAsFi=off
  Triggered To Workspace1 : dspsnks4/Triggered To Workspace  TriggerType=Falling edge  VariableName=Iin_Pulse_UP  Buffer=1000  Save2DMode=2-D array (concatenate along first dimension)
      settings: FixptAsFi=off
  Triggered To Workspace2 : dspsnks4/Triggered To Workspace  Commented=on  TriggerType=Falling edge  VariableName=PWM_T_DOWN  Buffer=1000  Save2DMode=2-D array (concatenate along first dimension)
      settings: FixptAsFi=off
  Triggered To Workspace3 : dspsnks4/Triggered To Workspace  TriggerType=Falling edge  VariableName=Iin_Pulse_DOWN  Buffer=1000  Save2DMode=2-D array (concatenate along first dimension)
      settings: FixptAsFi=off
  Triggered To Workspace4 : dspsnks4/Triggered To Workspace  TriggerType=Falling edge  VariableName=Iin_Pulse_UP_ref  Buffer=1000  Save2DMode=2-D array (concatenate along first dimension)
      settings: FixptAsFi=off
  Triggered To Workspace5 : dspsnks4/Triggered To Workspace  TriggerType=Falling edge  VariableName=Iin_Pulse_DOWN_ref  Buffer=1000  Save2DMode=2-D array (concatenate along first dimension)
      settings: FixptAsFi=off
  Unit Delay : UnitDelay  Commented=on  SampleTime=-1  HasFrameUpgradeWarning=on
  Unit Delay{1..2,4..5} (4 alike) : UnitDelay  SampleTime=-1  HasFrameUpgradeWarning=on
  Unit Delay3 : UnitDelay  Commented=on  SampleTime=-1  HasFrameUpgradeWarning=on
  Voltage Measurement{2,7,10..11} (4 alike) : spsVoltageMeasurementLib/Voltage Measurement  PhasorSimulation=off  OutputType=Complex  PSBequivalent=0
  Zero-Order Hold : ZeroOrderHold  SampleTime=1e-5
  Zero-Order Hold1 : ZeroOrderHold  SampleTime=1e-5
  powergui : spspowerguiLib/powergui  Priority=1  SimulationMode=Discrete  SampleTime=1e-7  frequency=60  Iterations=50  frequencyindice=0  Pbase=100e6  ErrMax=1e-4  UnitsV=kV  UnitsW=MW  buscounter=0  FunctionMessages=off  echomessages=off  EnableUseOfTLC=off  CurrentSourceSwitches=off  DisableSnubberDevices=off  DisableRonSwitches=off  DisableVfSwitches=off  DisplayEquations=off  AutomaticDiscreteSolvers=off  SolverType=Tustin/Backward Euler (TBE)  Interpol=off  ExternalGateDelay=off  methode=off  Ts=100  x0status=blocks  SPID=on  SwTol=0  HookPort=off  NonlinearTolerance=1e-4  nMaxIteration=100  ContinueOnMaxIteration=off  RestoreLinks=warning  ResistiveCurrentMeasurement=off  Frange=[0:2:500]  Ylog=off  Xlog=on  ShowGrid=off  save=off  variable=ZData  structure=0  ZoomFFT=off  StartTime=0.0  cycles=1  DisplayStyle=1  fundamental=60  FreqAxis=off  MaxFrequency=1000  frequencyindicesteady=1  RmsSteady=1  display=off
  状态判断 : Subsystem
  理想脉冲输出 : Subsystem  Commented=on
  tag scope: Down=global, State1=global, State=global, Up=global, io=global
  wires:
  [PWM2] -> Mosfet4/1
  Current Measurement12/1 -> Scope19/1, [IL2]
  [PWM4] -> Mosfet3/1
  Current Measurement11/1 -> Scope18/1, [IL1]
  Voltage Measurement10/1 -> Scope21/1, [VG1]
  [PWM1] -> Mosfet2/1
  Voltage Measurement11/1 -> Scope22/1, [VC2]
  Current Measurement8/1 -> [IB2]
  Current Measurement2/1 -> Scope11/1, [io]
  [VC1] -> Analog Filter Design2/1
  Analog Filter Design2/1 -> Sum5/1
  Sum5/1 -> PID Controller1/1
  Repeating Sequence2/1 -> Relational Operator2/2
  Constant4/1 -> Sum5/2
  [PWM3] -> Mosfet1/1
  Current Measurement1/1 -> Scope9/1
  Current Measurement3/1 -> [Iin]
  PID Controller3/1 -> Saturation1/1
  Sum1/1 -> PID Controller3/1
  PID Controller1/1 -> Scope29/1, Sum7/1
  [io] -> Sum6/1
  Sum7/1 -> Scope30/1, Sum1/1
  Sum6/1 -> Product/2
  Product/1 -> Sum7/2
  Constant6/1 -> Product/1
  [IL1] -> Sum1/2
  Constant8/1 -> Sum6/2
  Current Measurement/1 -> [I1]
  Current Measurement4/1 -> [I2]
  Current Measurement6/1 -> [IC1]
  Current Measurement7/1 -> [IC2]
  Repeating Sequence3/1 -> Controlled Current Source/1
  Current Measurement5/1 -> [IB1]
  Voltage Measurement7/1 -> Scope23/1, [VC1]
  Voltage Measurement2/1 -> [VG2], Scope16/1
  Subsystem1/2(Out2) -> [PWM2]
  From62/1 -> Subsystem1/5(In6)
  From51/1 -> Subsystem1/4(In5)
  [State] -> Subsystem1/6(In3)
  From50/1 -> Subsystem1/2(In2)
  From49/1 -> Subsystem1/1(In1)
  Subsystem1/1(Out1) -> [PWM1]
  Saturation3/1 -> Zero-Order Hold1/1
  Subsystem2/1(Out1) -> [PWM3]
  From70/1 -> Subsystem2/1(In1)
  From74/1 -> Subsystem2/2(In2)
  [State] -> Subsystem2/6(In3)
  From75/1 -> Subsystem2/4(In5)
  From77/1 -> Subsystem2/5(In6)
  Subsystem2/2(Out2) -> [PWM4]
  Constant11/1 -> Sum13/2
  [IL2] -> Sum11/2
  Constant9/1 -> Product3/1
  Product3/1 -> Sum14/2
  Sum13/1 -> Product3/2
  Sum14/1 -> Sum11/1
  [io] -> Sum13/1
  PID Controller4/1 -> Sum14/1
  Sum11/1 -> PID Controller5/1
  PID Controller5/1 -> Saturation3/1
  Constant3/1 -> Sum12/2
  Repeating Sequence1/1 -> Relational Operator3/2
  Sum12/1 -> PID Controller4/1
  Analog Filter Design3/1 -> Sum12/1
  [VC2] -> Analog Filter Design3/1
  Saturation1/1 -> Zero-Order Hold/1
  Zero-Order Hold/1 -> Relational Operator2/1
  Zero-Order Hold1/1 -> Relational Operator3/1
  From21/1 -> Scope12/1
  [io] -> Scope7/1
  Analog Filter Design12/1 -> Scope13/4
  From36/1 -> Sum9/2
  From15/1 -> Scope8/1
  From28/1 -> Analog Filter Design12/1
  [PWM4] -> Scope15/5
  [VG1] -> Scope7/5
  From48/1 -> Scope6/2
  From14/1 -> Scope10/4
  Analog Filter Design/1 -> Scope6/1
  From29/1 -> Sum/1
  From38/1 -> Scope6/3
  [VC1] -> Scope7/3
  From/1 -> Scope10/2
  From27/1 -> Analog Filter Design11/1
  From37/1 -> Scope14/3
  [PWM2] -> Scope15/3
  From39/1 -> Scope6/4
  [Iin] -> Analog Filter Design1/1, Analog Filter Design13/1
  Analog Filter Design1/1 -> Scope17/3, [Iin_f2]
  [io] -> Scope15/1
  Sum/1 -> Scope14/1
  From23/1 -> Scope12/3
  Analog Filter Design5/1 -> Scope8/2
  [PWM3] -> Scope15/4
  From24/1 -> Scope12/4
  [VG2] -> Scope7/4
  From26/1 -> Scope13/3
  From22/1 -> Analog Filter Design9/1
  From41/1 -> Sum10/2
  [VC2] -> Scope7/2
  Sum10/1 -> Analog Filter Design10/1
  From40/1 -> Sum10/1
  Analog Filter Design9/1 -> Scope12/2
  From9/1 -> Scope10/3
  From34/1 -> Sum/2
  From18/1 -> Analog Filter Design6/1
  Analog Filter Design13/1 -> Scope17/2, [Iin_f1]
  From46/1 -> Analog Filter Design/1
  Analog Filter Design6/1 -> Scope8/4
  [io] -> Scope17/1
  [PWM1] -> Scope15/2
  Sum9/1 -> Scope14/2
  Analog Filter Design11/1 -> Scope13/2
  Analog Filter Design10/1 -> Scope14/4
  [Iin] -> Scope10/1
  From35/1 -> Sum9/1
  From16/1 -> Scope8/3
  From25/1 -> Scope13/1
  From17/1 -> Analog Filter Design5/1
  On Delay5/1 -> OR5/2
  Unit Delay1/1 -> Triggered To Workspace1/1
  Discrete-Time Integrator2/1 -> Unit Delay2/1
  On Delay1/1 -> OR1/2
  Product4/1 -> Discrete-Time Integrator2/1, Scope1/1
  OR/1 -> Product1/1, Triggered To Workspace1/Trigger, Discrete-Time Integrator1/2
  Discrete-Time Integrator5/1 -> Unit Delay5/1
  [Iin_f2] -> Product5/2
  Unit Delay4/1 -> Triggered To Workspace4/1
  OR5/1 -> Product5/1, Discrete-Time Integrator5/2, Triggered To Workspace5/Trigger
  Product5/1 -> Scope1/2, Discrete-Time Integrator5/1
  Unit Delay2/1 -> Triggered To Workspace3/1
  [Iin_f1] -> Product4/2
  Discrete-Time Integrator4/1 -> Unit Delay4/1
  OR4/1 -> Discrete-Time Integrator4/2, Triggered To Workspace4/Trigger, Product2/1
  [Down] -> OR1/1, On Delay1/1
  Product2/1 -> Scope/2, Discrete-Time Integrator4/1
  Unit Delay5/1 -> Triggered To Workspace5/1
  [Iin_f1] -> Product1/2
  OR1/1 -> Triggered To Workspace3/Trigger, Discrete-Time Integrator2/2, Product4/1
  [Up] -> OR4/1, On Delay4/1
  On Delay4/1 -> OR4/2
  [Down] -> On Delay5/1, OR5/1
  On Delay/1 -> OR/2
  Product1/1 -> Discrete-Time Integrator1/1, Scope/1
  Discrete-Time Integrator1/1 -> Unit Delay1/1
  [Iin_f2] -> Product2/2
  [Up] -> On Delay/1, OR/1
  From92/1 -> Product8/1
  Product9/1 -> Subsystem8/1(In1)
  On Delay9/1 -> OR2/2
  From60/1 -> Subsystem11/1(In)
  From89/1 -> Product6/1
  Delay One Step7/1 -> Product8/2
  From90/1 -> Product7/1
  From67/1 -> Subsystem10/1(In)
  Delay One Step2/1 -> AND4/2
  Unit Delay3/1 -> Triggered To Workspace2/1
  AND4/1 -> Discrete-Time Integrator3/2, Triggered To Workspace2/Trigger, Discrete-Time Integrator3/1
  OR3/1 -> AND5/1
  Divide1/1 -> Unit Delay3/1
  Delay One Step8/1 -> Product9/2
  AND2/1 -> Triggered To Workspace/Trigger, Discrete-Time Integrator/2, Discrete-Time Integrator/1
  AND8/1 -> Subsystem5/1(In1)
  On Delay3/1 -> OR3/2
  Product7/1 -> Subsystem6/1(In1)
  Unit Delay/1 -> Triggered To Workspace/1
  Subsystem11/1(Out) -> OR2/1, On Delay9/1
  Discrete-Time Integrator/1 -> Divide/1
  OR2/1 -> AND8/1
  From94/1 -> Product9/1
  From87/1 -> Delay One Step5/1
  Subsystem9/1(Out) -> OR3/1, On Delay3/1
  From82/1 -> Subsystem/1(In)
  From66/1 -> Delay One Step3/1
  From10/1 -> Delay One Step2/1
  From91/1 -> Delay One Step7/1
  Discrete-Time Integrator3/1 -> Divide1/1
  Constant/1 -> Divide/2
  Delay One Step5/1 -> Product6/2
  From93/1 -> Delay One Step8/1
  Divide/1 -> Unit Delay/1
  From61/1 -> Delay One Step1/1
  Delay One Step6/1 -> Product7/2
  Subsystem/1(Out) -> AND4/1
  Product6/1 -> Subsystem3/1(In1)
  Subsystem10/1(Out) -> AND2/1
  Product8/1 -> Subsystem7/1(In1)
  From55/1 -> Delay One Step4/1
  From88/1 -> Delay One Step6/1
  AND5/1 -> Subsystem4/1(In1)
  Delay One Step4/1 -> AND8/2
  From68/1 -> Subsystem9/1(In)
  Delay One Step3/1 -> AND2/2
  Constant5/1 -> Divide1/2
  Delay One Step1/1 -> AND5/2
  Add/1 -> Math Function/1
  [io] -> 状态判断/1(In1)
  From73/1 -> Relational Operator5/1
  From59/1 -> NOT8/1
  From65/1 -> Add/1
  状态判断/1(y) -> [Up]
  Subsystem13/1(Out) -> AND9/2
  状态判断/3(Out3) -> [Down]
  From56/1 -> On Delay12/1
  On Delay8/1 -> AND3/1
  On Delay11/1 -> AND9/1
  AND3/1 -> Subsystem14/1(In)
  Relational Operator/1 -> AND1/2
  [Down] -> Subsystem13/1(In)
  NOT8/1 -> AND7/2
  From69/1 -> On Delay2/1
  [Up] -> On Delay11/1
  From71/1 -> Relational Operator/1
  AND6/1 -> Goto16/1
  NOT7/1 -> AND6/2
  From58/1 -> On Delay10/1
  Clock/1 -> Triggered Subsystem/1(In1), [t]
  Constant1/1 -> Math Function/2
  [State1] -> Triggered Subsystem/Trigger
  Constant10/1 -> Relational Operator5/2
  Triggered Subsystem/1(Out1) -> [t0]
  On Delay2/1 -> AND1/1
  From72/1 -> On Delay8/1
  状态判断/2(Out2) -> [State]
  AND7/1 -> Goto17/1
  AND1/1 -> Goto23/1
  From57/1 -> NOT7/1
  Math Function/1 -> Goto24/1
  AND9/1 -> [State1]
  On Delay10/1 -> AND7/1
  On Delay12/1 -> AND6/1
  Relational Operator5/1 -> AND3/2
  From63/1 -> Add/2
  Constant2/1 -> Relational Operator/2
  Relational Operator2/1 -> Delay One Step/1
  Delay One Step/1 -> Subsystem1/3(In)
  Relational Operator3/1 -> Delay One Step9/1
  Delay One Step9/1 -> Subsystem2/3(In)
  Subsystem14/1(Out) -> Goto22/1
  MATLAB Function5/2(Q_sync) -> Goto37/1
  Constant26/1 -> Sum18/2
  From113/1 -> Sum18/1
  From112/1 -> MATLAB Function5/2(Vo)
  MATLAB Function5/1(Q_main) -> Goto36/1
  Sum17/1 -> Product13/2
  Constant24/1 -> MATLAB Function4/1(Vref)
  MATLAB Function4/1(Q_main) -> Goto25/1
  Product14/1 -> MATLAB Function5/3(Iref_ext)
  From111/1 -> MATLAB Function4/4(iL)
  Product13/1 -> MATLAB Function4/3(Iref_ext)
  Constant22/1 -> Product13/1
  Constant23/1 -> Sum17/2
  Sum18/1 -> Product14/2
  MATLAB Function4/2(Q_sync) -> Goto26/1
  Constant27/1 -> MATLAB Function5/1(Vref)
  From109/1 -> MATLAB Function4/2(Vo)
  Constant25/1 -> Product14/1
  From110/1 -> Sum17/1
  From114/1 -> MATLAB Function5/4(iL)
  MATLAB Function6/3(Flag_on_time) -> Divide2/1, Scope26/2
  MATLAB Function6/1(PWM_gated) -> Scope26/1
  [Down] -> Subsystem15/1(In)
  MATLAB Function7/1(PWM_gated) -> Scope27/1
  MATLAB Function7/3(Flag_on_time) -> Divide3/1, Scope27/2
  [PWM1] -> MATLAB Function7/2(PWM)
  [PWM1] -> MATLAB Function6/2(PWM)
  Constant7/1 -> Divide2/2
  Divide3/1 -> Scope27/3, To Workspace1/1
  Constant12/1 -> Divide3/2
  Divide2/1 -> Scope26/3, To Workspace/1
  [Up] -> Subsystem12/1(In)
  Subsystem12/1(Out) -> MATLAB Function6/1(Flag)
  Subsystem15/1(Out) -> MATLAB Function7/1(Flag)
  connections:
  Series RL Branch1/RConn1 -- Voltage Measurement7/LConn2 -- DC Voltage Source1/LConn1 -- Mosfet4/RConn1 -- Voltage Measurement10/LConn2 -- Current Measurement2/LConn1 -- Series RLC Branch2/RConn1
  Current Measurement8/RConn1 -- Current Measurement3/LConn1 -- Mosfet3/LConn1 -- Current Measurement1/RConn1 -- Voltage Measurement11/LConn1 -- Series RLC Branch18/LConn1
  Current Measurement12/RConn1 -- Mosfet3/RConn1 -- Mosfet1/LConn1
  Current Measurement11/RConn1 -- Series RLC Branch20/LConn1
  Series RLC Branch20/RConn1 -- Current Measurement7/LConn1 -- Current Measurement4/LConn1
  Current Measurement12/LConn1 -- Series RLC Branch19/RConn1
  Series RLC Branch19/LConn1 -- Voltage Measurement11/LConn2 -- Current Measurement/RConn1 -- Current Measurement6/RConn1
  Series RLC Branch1/LConn1 -- Current Measurement8/LConn1 -- Voltage Measurement2/LConn1
  Current Measurement2/RConn1 -- Controlled Current Source/LConn1
  Current Measurement1/LConn1 -- Controlled Current Source/RConn1
  Current Measurement3/RConn1 -- DC Voltage Source1/RConn1
  Current Measurement5/LConn1 -- Series RLC Branch2/LConn1
  Current Measurement4/RConn1 -- Mosfet1/RConn1 -- Voltage Measurement2/LConn2 -- Series RLC Branch1/RConn1
  Current Measurement7/RConn1 -- Voltage Measurement7/LConn1 -- Series RL Branch1/LConn1
  Series RLC Branch18/RConn1 -- Current Measurement6/LConn1
  Mosfet4/LConn1 -- Mosfet2/RConn1 -- Current Measurement11/LConn1
  Current Measurement/LConn1 -- Current Measurement5/RConn1 -- Voltage Measurement10/LConn1 -- Mosfet2/LConn1

== system DualBuckPPS22016/Subsystem ==
  In : Inport
  On Delay10 : spsOnDelayLib/On Delay  DelayType=On delay  delay=ceil(TP*1e5)*1e-5-TP  ic=0  Ts=0
  On Delay11 : spsOnDelayLib/On Delay  DelayType=Off delay  delay=ceil((TP-(ceil(TP*1e5)*1e-5-TP))*1e5)*1e-5-(TP-(ceil(TP*1e5)*1e-5-TP))  ic=0  Ts=0
  Out : Outport
  wires:
  On Delay10/1 -> On Delay11/1
  In/1 -> On Delay10/1
  On Delay11/1 -> Out/1

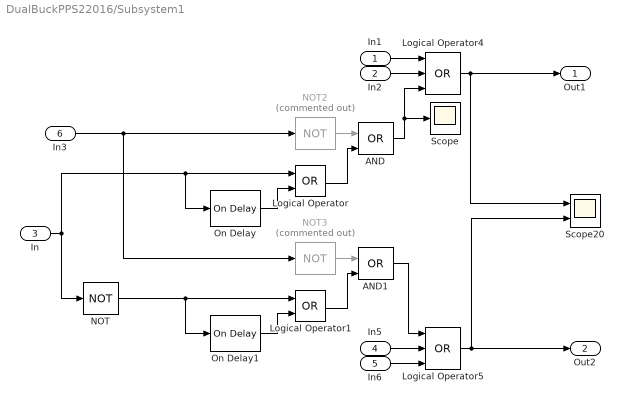
== system DualBuckPPS22016/Subsystem1 ==
  In1 : Inport
  In2 : Inport  Port=2
  In : Inport  Port=3
  In5 : Inport  Port=4
  In6 : Inport  Port=5
  In3 : Inport  Port=6
  AND : Logic  Operator=OR  IconShape=distinctive  AllPortsSameDT=off  OutDataTypeStr=boolean
  AND1 : Logic  Operator=OR  IconShape=distinctive  AllPortsSameDT=off  OutDataTypeStr=boolean
  Logical Operator : Logic  Operator=OR  AllPortsSameDT=off  OutDataTypeStr=boolean
  Logical Operator1 : Logic  Operator=OR  AllPortsSameDT=off  OutDataTypeStr=boolean
  Logical Operator4 : Logic  Operator=OR  Inputs=3  AllPortsSameDT=off  OutDataTypeStr=boolean
  Logical Operator5 : Logic  Operator=OR  Inputs=3  AllPortsSameDT=off  OutDataTypeStr=boolean
  NOT : Logic  Operator=NOT  IconShape=distinctive  AllPortsSameDT=off  OutDataTypeStr=boolean
  NOT2 : Logic  Commented=on  Operator=NOT  IconShape=distinctive  AllPortsSameDT=off  OutDataTypeStr=boolean
  NOT3 : Logic  Commented=on  Operator=NOT  IconShape=distinctive  AllPortsSameDT=off  OutDataTypeStr=boolean
  On Delay : spsOnDelayLib/On Delay  DelayType=On delay  delay=100e-9  ic=0  Ts=0
  On Delay1 : spsOnDelayLib/On Delay  DelayType=On delay  delay=100e-9  ic=0  Ts=0
  Scope : Scope
  Scope20 : Scope  NumInputPorts=2
  Out1 : Outport
  Out2 : Outport  Port=2
  wires:
  In5/1 -> Logical Operator5/2
  In6/1 -> Logical Operator5/3
  In3/1 -> NOT3/1, NOT2/1
  In/1 -> Logical Operator/1, On Delay/1, NOT/1
  NOT2/1 -> AND/1
  NOT3/1 -> AND1/1
  Logical Operator1/1 -> AND1/2
  NOT/1 -> Logical Operator1/1, On Delay1/1
  Logical Operator5/1 -> Scope20/2, Out2/1
  Logical Operator4/1 -> Scope20/1, Out1/1
  In2/1 -> Logical Operator4/2
  On Delay/1 -> Logical Operator/2
  On Delay1/1 -> Logical Operator1/2
  AND1/1 -> Logical Operator5/1
  AND/1 -> Logical Operator4/3, Scope/1
  Logical Operator/1 -> AND/2
  In1/1 -> Logical Operator4/1

== system DualBuckPPS22016/Subsystem10 ==
  In : Inport
  On Delay10 : spsOnDelayLib/On Delay  DelayType=On delay  delay=10e-6  ic=0  Ts=0
  On Delay11 : spsOnDelayLib/On Delay  DelayType=Off delay  delay=ceil(TP*1e5)*1e-5-TP  ic=0  Ts=0
  Out : Outport
  wires:
  On Delay11/1 -> Out/1
  In/1 -> On Delay10/1
  On Delay10/1 -> On Delay11/1

== system DualBuckPPS22016/Subsystem11 ==
  In : Inport
  On Delay10 : spsOnDelayLib/On Delay  DelayType=On delay  delay=ceil(TP*1e5)*1e-5-TP  ic=0  Ts=0
  On Delay11 : spsOnDelayLib/On Delay  DelayType=Off delay  delay=ceil((TP-(ceil(TP*1e5)*1e-5-TP))*1e5)*1e-5-(TP-(ceil(TP*1e5)*1e-5-TP))  ic=0  Ts=0
  Out : Outport
  wires:
  On Delay10/1 -> On Delay11/1
  In/1 -> On Delay10/1
  On Delay11/1 -> Out/1

== system DualBuckPPS22016/Subsystem12 ==
  In : Inport
  On Delay10 : spsOnDelayLib/On Delay  DelayType=On delay  delay=1e-5  ic=0  Ts=0
  On Delay2 : spsOnDelayLib/On Delay  DelayType=Off delay  delay=1e-5  ic=0  Ts=0
  Out : Outport
  wires:
  On Delay2/1 -> Out/1
  In/1 -> On Delay10/1
  On Delay10/1 -> On Delay2/1

== system DualBuckPPS22016/Subsystem13 ==
  In : Inport
  On Delay10 : spsOnDelayLib/On Delay  DelayType=On delay  delay=ceil(TP*1e5)*1e-5-TP  ic=0  Ts=0
  On Delay2 : spsOnDelayLib/On Delay  DelayType=Off delay  delay=ceil((TP-(ceil(TP*1e5)*1e-5-TP))*1e5)*1e-5-(TP-(ceil(TP*1e5)*1e-5-TP))  ic=0  Ts=0
  Out : Outport
  wires:
  On Delay10/1 -> On Delay2/1
  In/1 -> On Delay10/1
  On Delay2/1 -> Out/1

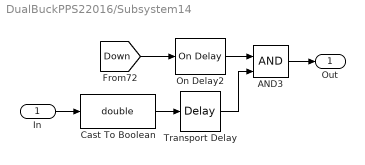
== system DualBuckPPS22016/Subsystem14 ==
  In : Inport
  AND3 : Logic  IconShape=distinctive  AllPortsSameDT=off  OutDataTypeStr=boolean
  Cast To Boolean : DataTypeConversion  OutDataTypeStr=double  SaturateOnIntegerOverflow=off  RndMeth=Floor
  On Delay2 : spsOnDelayLib/On Delay  DelayType=Off delay  delay=ceil((TP-(ceil(TP*1e5)*1e-5-TP))*1e5)*1e-5-(TP-(ceil(TP*1e5)*1e-5-TP))  ic=0  Ts=0
  Transport Delay : TransportDelay  DelayTime=ceil(TP*1e5)*1e-5-TP
  Out : Outport
  wires:
  Transport Delay/1 -> AND3/2
  In/1 -> Cast To Boolean/1
  Cast To Boolean/1 -> Transport Delay/1
  On Delay2/1 -> AND3/1
  [Down] -> On Delay2/1
  AND3/1 -> Out/1

== system DualBuckPPS22016/Subsystem15 ==
  In : Inport
  On Delay10 : spsOnDelayLib/On Delay  DelayType=On delay  delay=1e-5  ic=0  Ts=0
  On Delay2 : spsOnDelayLib/On Delay  DelayType=Off delay  delay=1e-5  ic=0  Ts=0
  Out : Outport
  wires:
  On Delay10/1 -> On Delay2/1
  In/1 -> On Delay10/1
  On Delay2/1 -> Out/1

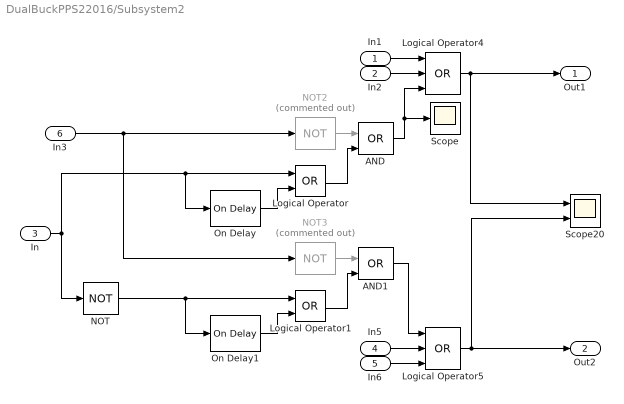
== system DualBuckPPS22016/Subsystem2 ==
  In1 : Inport
  In2 : Inport  Port=2
  In : Inport  Port=3
  In5 : Inport  Port=4
  In6 : Inport  Port=5
  In3 : Inport  Port=6
  AND : Logic  Operator=OR  IconShape=distinctive  AllPortsSameDT=off  OutDataTypeStr=boolean
  AND1 : Logic  Operator=OR  IconShape=distinctive  AllPortsSameDT=off  OutDataTypeStr=boolean
  Logical Operator : Logic  Operator=OR  AllPortsSameDT=off  OutDataTypeStr=boolean
  Logical Operator1 : Logic  Operator=OR  AllPortsSameDT=off  OutDataTypeStr=boolean
  Logical Operator4 : Logic  Operator=OR  Inputs=3  AllPortsSameDT=off  OutDataTypeStr=boolean
  Logical Operator5 : Logic  Operator=OR  Inputs=3  AllPortsSameDT=off  OutDataTypeStr=boolean
  NOT : Logic  Operator=NOT  IconShape=distinctive  AllPortsSameDT=off  OutDataTypeStr=boolean
  NOT2 : Logic  Commented=on  Operator=NOT  IconShape=distinctive  AllPortsSameDT=off  OutDataTypeStr=boolean
  NOT3 : Logic  Commented=on  Operator=NOT  IconShape=distinctive  AllPortsSameDT=off  OutDataTypeStr=boolean
  On Delay : spsOnDelayLib/On Delay  DelayType=On delay  delay=100e-9  ic=0  Ts=0
  On Delay1 : spsOnDelayLib/On Delay  DelayType=On delay  delay=100e-9  ic=0  Ts=0
  Scope : Scope
  Scope20 : Scope  NumInputPorts=2
  Out1 : Outport
  Out2 : Outport  Port=2
  wires:
  In1/1 -> Logical Operator4/1
  Logical Operator/1 -> AND/2
  AND/1 -> Scope/1, Logical Operator4/3
  AND1/1 -> Logical Operator5/1
  On Delay1/1 -> Logical Operator1/2
  On Delay/1 -> Logical Operator/2
  In2/1 -> Logical Operator4/2
  Logical Operator4/1 -> Out1/1, Scope20/1
  Logical Operator5/1 -> Out2/1, Scope20/2
  NOT/1 -> On Delay1/1, Logical Operator1/1
  Logical Operator1/1 -> AND1/2
  NOT3/1 -> AND1/1
  NOT2/1 -> AND/1
  In/1 -> NOT/1, On Delay/1, Logical Operator/1
  In3/1 -> NOT2/1, NOT3/1
  In6/1 -> Logical Operator5/3
  In5/1 -> Logical Operator5/2

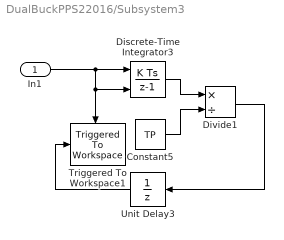
== system DualBuckPPS22016/Subsystem3 ==
  In1 : Inport
  Constant5 : Constant  Value=TP
  Discrete-Time Integrator3 : DiscreteIntegrator  ExternalReset=falling  SampleTime=-1  ICPrevOutput=DiscIntNeverNeededParam  ICPrevScaledInput=DiscIntNeverNeededParam
  Divide1 : Product  Inputs=*/
  Triggered To Workspace1 : dspsnks4/Triggered To Workspace  TriggerType=Falling edge  VariableName=VC1_UP  Buffer=1000  Save2DMode=2-D array (concatenate along first dimension)
      settings: FixptAsFi=off
  Unit Delay3 : UnitDelay  SampleTime=-1  HasFrameUpgradeWarning=on
  wires:
  Divide1/1 -> Unit Delay3/1
  Constant5/1 -> Divide1/2
  In1/1 -> Triggered To Workspace1/Trigger, Discrete-Time Integrator3/2, Discrete-Time Integrator3/1
  Discrete-Time Integrator3/1 -> Divide1/1
  Unit Delay3/1 -> Triggered To Workspace1/1

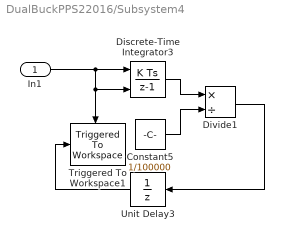
== system DualBuckPPS22016/Subsystem4 ==
  In1 : Inport
  Constant5 : Constant  Value=1/100000
  Discrete-Time Integrator3 : DiscreteIntegrator  ExternalReset=falling  SampleTime=-1  ICPrevOutput=DiscIntNeverNeededParam  ICPrevScaledInput=DiscIntNeverNeededParam
  Divide1 : Product  Inputs=*/
  Triggered To Workspace1 : dspsnks4/Triggered To Workspace  TriggerType=Falling edge  VariableName=PWM_S_UP  Buffer=1000  Save2DMode=2-D array (concatenate along first dimension)
      settings: FixptAsFi=off
  Unit Delay3 : UnitDelay  SampleTime=-1  HasFrameUpgradeWarning=on
  wires:
  Divide1/1 -> Unit Delay3/1
  Constant5/1 -> Divide1/2
  In1/1 -> Triggered To Workspace1/Trigger, Discrete-Time Integrator3/2, Discrete-Time Integrator3/1
  Discrete-Time Integrator3/1 -> Divide1/1
  Unit Delay3/1 -> Triggered To Workspace1/1
